simulink model "SoftGripperScene3D"  (R2026b)
settings: Solver=FixedStepDiscrete  StopTime=replay.tEnd  FixedStep=replay.Ts
undefined symbols (not defined in the file): replay, Sim3dSensor
libraries: sim3dlib x6, robotsim3dlib x5, sim3dcameralib x1
settings Model: Creator=amavromm  LastModifiedBy=amavromm

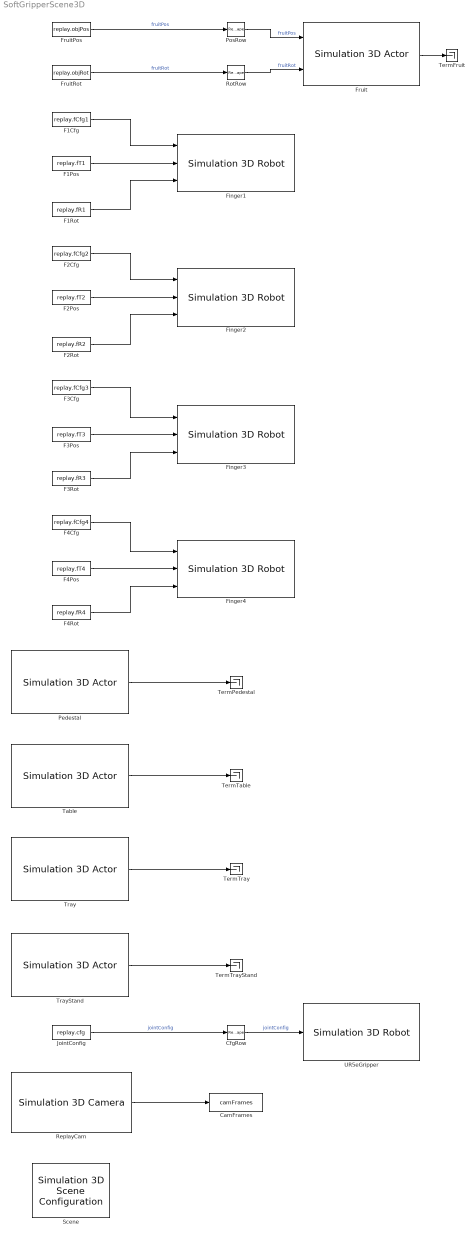
== system SoftGripperScene3D ==
  CamFrames : ToWorkspace  VariableName=camFrames  SaveFormat=Timeseries  SampleTime=-1
  CfgRow : Reshape  OutputDimensionality=Customize  OutputDimensions=[1 6]
  F1Cfg : FromWorkspace  VariableName=replay.fCfg1  OutputAfterFinalValue=Holding final value
  F1Pos : FromWorkspace  VariableName=replay.fT1  OutputAfterFinalValue=Holding final value
  F1Rot : FromWorkspace  VariableName=replay.fR1  OutputAfterFinalValue=Holding final value
  F2Cfg : FromWorkspace  VariableName=replay.fCfg2  OutputAfterFinalValue=Holding final value
  F2Pos : FromWorkspace  VariableName=replay.fT2  OutputAfterFinalValue=Holding final value
  F2Rot : FromWorkspace  VariableName=replay.fR2  OutputAfterFinalValue=Holding final value
  F3Cfg : FromWorkspace  VariableName=replay.fCfg3  OutputAfterFinalValue=Holding final value
  F3Pos : FromWorkspace  VariableName=replay.fT3  OutputAfterFinalValue=Holding final value
  F3Rot : FromWorkspace  VariableName=replay.fR3  OutputAfterFinalValue=Holding final value
  F4Cfg : FromWorkspace  VariableName=replay.fCfg4  OutputAfterFinalValue=Holding final value
  F4Pos : FromWorkspace  VariableName=replay.fT4  OutputAfterFinalValue=Holding final value
  F4Rot : FromWorkspace  VariableName=replay.fR4  OutputAfterFinalValue=Holding final value
  Finger1 : robotsim3dlib/Simulation 3D Robot  actorInputType=RigidBodyTree Object  RigidBodyTree=replay.fingerTree  ActorName=Finger1  existActorChekBox=off  initialTrans=replay.fT0(1,:)  initialRot=replay.fR0(1,:)  initialConfig=replay.fCfg0  EndEffector=link8  eeOffsetInpChekBox=off  eeTargetTrans=[0 0 0]  eeTargetRot=[0 0 0]  enableRegionGraspChekBox=off  regionGraspInpChekBox=off  eeTargTransDiff=[0.2 0.2 0.2]  eeTargRotDiff=[0 0 0]  enableVisualVisualization=on  enableCollisionVisualization=off  collisionGeomColor=[0 1 0]  collisionGeomTransp=0.1  inpConfEnbVal=on  inpGraspEnbVal=off  inpTransEnbVal=on  outConfEnbVal=off  outGraspEnbVal=off  outTransEnbVal=off  SampleTime=replay.Ts  ActorType=SimulinkVehicle  ID=C  aMode=6  ActorTag=Finger1  Mesh=RigidBodyTree
  Finger2 : robotsim3dlib/Simulation 3D Robot  actorInputType=RigidBodyTree Object  RigidBodyTree=replay.fingerTree  ActorName=Finger2  existActorChekBox=off  initialTrans=replay.fT0(2,:)  initialRot=replay.fR0(2,:)  initialConfig=replay.fCfg0  EndEffector=link8  eeOffsetInpChekBox=off  eeTargetTrans=[0 0 0]  eeTargetRot=[0 0 0]  enableRegionGraspChekBox=off  regionGraspInpChekBox=off  eeTargTransDiff=[0.2 0.2 0.2]  eeTargRotDiff=[0 0 0]  enableVisualVisualization=on  enableCollisionVisualization=off  collisionGeomColor=[0 1 0]  collisionGeomTransp=0.1  inpConfEnbVal=on  inpGraspEnbVal=off  inpTransEnbVal=on  outConfEnbVal=off  outGraspEnbVal=off  outTransEnbVal=off  SampleTime=replay.Ts  ActorType=SimulinkVehicle  ID=C  aMode=6  ActorTag=Finger2  Mesh=RigidBodyTree
  Finger3 : robotsim3dlib/Simulation 3D Robot  actorInputType=RigidBodyTree Object  RigidBodyTree=replay.fingerTree  ActorName=Finger3  existActorChekBox=off  initialTrans=replay.fT0(3,:)  initialRot=replay.fR0(3,:)  initialConfig=replay.fCfg0  EndEffector=link8  eeOffsetInpChekBox=off  eeTargetTrans=[0 0 0]  eeTargetRot=[0 0 0]  enableRegionGraspChekBox=off  regionGraspInpChekBox=off  eeTargTransDiff=[0.2 0.2 0.2]  eeTargRotDiff=[0 0 0]  enableVisualVisualization=on  enableCollisionVisualization=off  collisionGeomColor=[0 1 0]  collisionGeomTransp=0.1  inpConfEnbVal=on  inpGraspEnbVal=off  inpTransEnbVal=on  outConfEnbVal=off  outGraspEnbVal=off  outTransEnbVal=off  SampleTime=replay.Ts  ActorType=SimulinkVehicle  ID=C  aMode=6  ActorTag=Finger3  Mesh=RigidBodyTree
  Finger4 : robotsim3dlib/Simulation 3D Robot  actorInputType=RigidBodyTree Object  RigidBodyTree=replay.fingerTree  ActorName=Finger4  existActorChekBox=off  initialTrans=replay.fT0(4,:)  initialRot=replay.fR0(4,:)  initialConfig=replay.fCfg0  EndEffector=link8  eeOffsetInpChekBox=off  eeTargetTrans=[0 0 0]  eeTargetRot=[0 0 0]  enableRegionGraspChekBox=off  regionGraspInpChekBox=off  eeTargTransDiff=[0.2 0.2 0.2]  eeTargRotDiff=[0 0 0]  enableVisualVisualization=on  enableCollisionVisualization=off  collisionGeomColor=[0 1 0]  collisionGeomTransp=0.1  inpConfEnbVal=on  inpGraspEnbVal=off  inpTransEnbVal=on  outConfEnbVal=off  outGraspEnbVal=off  outTransEnbVal=off  SampleTime=replay.Ts  ActorType=SimulinkVehicle  ID=C  aMode=6  ActorTag=Finger4  Mesh=RigidBodyTree
  Fruit : sim3dlib/Simulation 3D Actor  Priority=1  ActorName=Fruit  ParentName=Scene Origin  Operation=Create at setup  InitScriptText=|  SampleTime=replay.Ts  Translation=replay.objPos0  Rotation=[0 0 0]  Scale=[1 1 1]  InputsText=Fruit.Translation Fruit.Rotation  aMode=aMode  ActorTag=Fruit  ActorType=Sim3dActor  ID=C
      | createShape(Actor, 'sphere', [0.08 0.08 0.08]);
      | Actor.Color = [0.80 0.12 0.12];
      | Actor.Mobility = sim3d.utils.MobilityTypes.Movable;
  FruitPos : FromWorkspace  VariableName=replay.objPos  OutputAfterFinalValue=Holding final value
  FruitRot : FromWorkspace  VariableName=replay.objRot  OutputAfterFinalValue=Holding final value
  JointConfig : FromWorkspace  VariableName=replay.cfg  OutputAfterFinalValue=Holding final value
  Pedestal : sim3dlib/Simulation 3D Actor  Priority=1  ActorName=Pedestal  ParentName=Scene Origin  Operation=Create at setup  InitScriptText=|  SampleTime=-1  Translation=replay.pedestalT  Rotation=[0 0 0]  Scale=[1 1 1]  aMode=aMode  ActorTag=Pedestal  ActorType=Sim3dActor  ID=C
      | createShape(Actor, 'box', [0.25 0.25 0.75]);
      | Actor.Color = [0.35 0.35 0.38];
  PosRow : Reshape  OutputDimensionality=Customize  OutputDimensions=[1 3]
  ReplayCam : sim3dcameralib/Simulation 3D Camera  Priority=1  sensorTag=Sim3dSensor�  sensorId=1  sensorName=Sim3dSensor�  vehTagList={'<empty>';'Custom ...';'Finger1';'Fruit';'Pedestal';'Scene Origin';'SimulinkVehicle1';'SimulinkVehicle2';'SimulinkVehicle3';'Table';'Tray';'TrayStand';'UR5eGripper'}  vehTag=Scene Origin  CoordinateSystem=Default  mountLoc=Origin  offsetFlag=on  tmountOffset=replay.camT  extTmount=off  rmountOffset=replay.camR  extRmount=off  FocalLength=[330 330]  OpticalCenter=[240 180]  ImageSize=[360 480]  RadialDistortion=[0, 0]  TangentialDistortion=[0, 0]  SensorSkew=0  VisualizeFieldOfView=off  FieldOfViewRange=61  DepthOutportEnabled=off  SemanticOutportEnabled=off  TransformOutportEnabled=off  SampleTime=replay.camTs  mountPoint=[0.67 0.1 0.839]  mountOrientation=[0 -0.0671660950233252 -2.40377759346933]  aMode=aMode  ID=1
  RotRow : Reshape  OutputDimensionality=Customize  OutputDimensions=[1 3]
  Scene : sim3dlib/Simulation 3D Scene Configuration  Priority=0  EnableWindow=on  ViewerType=Default Viewer  ProjectFormat=Default Scenes  SceneDesc=Open surface  ProjectName=C:\Program Files\MATLAB\R2026b\toolbox\shared\sim3d_projects\automotive_project_windows\UE\WindowsNoEditor\VehicleSimulation.exe  ScenePath=/Game/Maps/HwStrght  EnableOpenDRIVE=off  vehTagList={'Custom';'Scene Origin'}  vehTag=Scene Origin  AttachedCameraRelativeTranslation=[0 0 0]  FreeCameraDefaultInitialTranslation=[-6, 0, 2]  AttachedCameraRelativeRotation=[0, -15, 0]  FreeCameraDefaultInitialRotation=[0, -15, 0]  ViewpointName=Custom  FreeCameraInitialTranslation=[0 0 0]  FreeCameraInitialRotation=[0 0 0]  OpVisEn=off  Ts=replay.Ts  EnableRemoteAccess=off  SimulationMode=CoSimulation  SimulateUsing=Interpreted execution  EnableAnimationRecording=off  OverrideDefaultRecording=off  AnimationRecordingFileName=sim3dAnimation.mat  AnimationRecordingInterval=[0 inf]  EnableWeather=off  SunAzimuth=90  SunAltitude=40.0  EnableGeospatialSun=off  Latitude=0  Longitude=0  Date=2023-01-01  Time=10:30:00  GeoTimeZone=-5.0  SunDaylightSaving=off  wind=1  clouds=10  EnableVolumetricClouds=off  CloudCoverage=0  CloudAltitude=6  fog=0  rain=0  RaindropsEffect=off  SnowDensity=0  EnableGeospatial=off  TilesetSource=Earth terrain  UseTrueOrigin=off  OriginHeight=200  OriginLatitude=40.744652  OriginLongitude=-73.988864  MapStyle=Aerial  AdditionalAssetIDs=[]  UseAdvancedSunSky=off  SolarTime=11  TimeZone=-5  Day=21  Month=9  Year=2022  UseDaylightSavingTime=on  DSTStartDay=10  DSTStartMonth=3  DSTEndDay=3  DSTEndMonth=11  DSTSwitchHour=2  sensorTag=MainCamera1  sensorId=1  sensorName=MainCamera1  mountLoc=Origin  offsetFlag=off  tmountOffset=[0, 0, 0]  rmountOffset=[0, 0, 0]  HorizontalResolution=1280  VerticalResolution=720  HorizontalFOV=60  mountPoint=[0 0 0]  mountOrientation=[0 0 0]  aMode=aMode  ID=1  GeoTrigger=Inactive  ViewNameList={'Custom'}  ViewTranslationList={'[0 0 0]'}  ViewRotationList={'[0 0 0]'}
  Table : sim3dlib/Simulation 3D Actor  Priority=1  ActorName=Table  ParentName=Scene Origin  Operation=Create at setup  InitScriptText=|  SampleTime=-1  Translation=replay.tableT  Rotation=[0 0 0]  Scale=[1 1 1]  aMode=aMode  ActorTag=Table  ActorType=Sim3dActor  ID=C
      | createShape(Actor, 'box', [0.30 0.30 0.02]);
      | Actor.Color = [0.55 0.40 0.28];
  TermFruit : Terminator
  TermPedestal : Terminator
  TermTable : Terminator
  TermTray : Terminator
  TermTrayStand : Terminator
  Tray : sim3dlib/Simulation 3D Actor  Priority=1  ActorName=Tray  ParentName=Scene Origin  Operation=Create at setup  InitScriptText=|  SampleTime=-1  Translation=replay.trayT  Rotation=[0 0 0]  Scale=[1 1 1]  aMode=aMode  ActorTag=Tray  ActorType=Sim3dActor  ID=C
      | createShape(Actor, 'box', [0.20 0.20 0.02]);
      | Actor.Color = [0.20 0.35 0.60];
  TrayStand : sim3dlib/Simulation 3D Actor  Priority=1  ActorName=TrayStand  ParentName=Scene Origin  Operation=Create at setup  InitScriptText=|  SampleTime=-1  Translation=replay.trayStandT  Rotation=[0 0 0]  Scale=[1 1 1]  aMode=aMode  ActorTag=TrayStand  ActorType=Sim3dActor  ID=C
      | createShape(Actor, 'box', [0.24 0.24 0.75]);
      | Actor.Color = [0.55 0.40 0.28];
  UR5eGripper : robotsim3dlib/Simulation 3D Robot  actorInputType=RigidBodyTree Object  RigidBodyTree=replay.tree  ActorName=UR5eGripper  existActorChekBox=off  initialTrans=replay.robotT  initialRot=[0 0 0]  initialConfig=replay.cfg0  EndEffector=tool0  eeOffsetInpChekBox=off  eeTargetTrans=[0 0 0]  eeTargetRot=[0 0 0]  enableRegionGraspChekBox=off  regionGraspInpChekBox=off  eeTargTransDiff=[0.2 0.2 0.2]  eeTargRotDiff=[0 0 0]  enableVisualVisualization=on  enableCollisionVisualization=off  collisionGeomColor=[0 1 0]  collisionGeomTransp=0.1  inpConfEnbVal=on  inpGraspEnbVal=off  inpTransEnbVal=off  outConfEnbVal=off  outGraspEnbVal=off  outTransEnbVal=off  SampleTime=replay.Ts  ActorType=SimulinkVehicle  ID=C  aMode=6  ActorTag=UR5eGripper  Mesh=RigidBodyTree
  wires:
  F4Rot/1 -> Finger4/3
  F4Pos/1 -> Finger4/2
  F4Cfg/1 -> Finger4/1
  F3Rot/1 -> Finger3/3
  F3Pos/1 -> Finger3/2
  F3Cfg/1 -> Finger3/1
  F2Rot/1 -> Finger2/3
  F2Pos/1 -> Finger2/2
  F2Cfg/1 -> Finger2/1
  F1Rot/1 -> Finger1/3
  F1Pos/1 -> Finger1/2
  F1Cfg/1 -> Finger1/1
  CfgRow/1 -> UR5eGripper/1  "jointConfig"
  RotRow/1 -> Fruit/2  "fruitRot"
  PosRow/1 -> Fruit/1  "fruitPos"
  FruitRot/1 -> RotRow/1  "fruitRot"
  FruitPos/1 -> PosRow/1  "fruitPos"
  JointConfig/1 -> CfgRow/1  "jointConfig"
  Fruit/1 -> TermFruit/1
  Table/1 -> TermTable/1
  Tray/1 -> TermTray/1
  ReplayCam/1 -> CamFrames/1
  Pedestal/1 -> TermPedestal/1
  TrayStand/1 -> TermTrayStand/1
